simulink model "structure_implement"  (R2026b)
settings: Solver=VariableStepAuto
undefined symbols (not defined in the file or in its folder): DiscIntNeverNeededParam, Ts
settings Model: Creator=aomar  LastModifiedBy=aomar

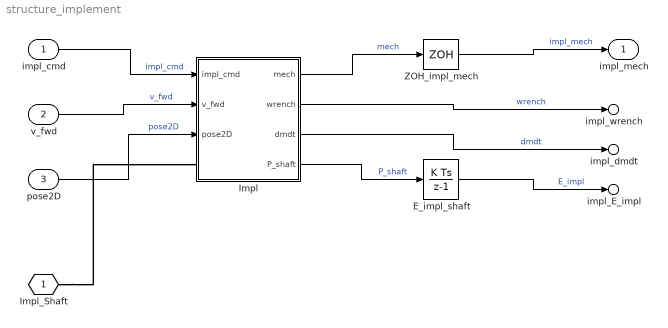
== system structure_implement ==
  impl_cmd : Inport  OutDataTypeStr=Bus: Bus_ImplementCmd  SampleTime=Ts.ctrl
  v_fwd : Inport  Port=2
  pose2D : Inport  Port=3
  E_impl_shaft : DiscreteIntegrator  gainval=1  SampleTime=Ts.base  ICPrevOutput=DiscIntNeverNeededParam  ICPrevScaledInput=DiscIntNeverNeededParam
  Impl : Subsystem  Variant=on
  ZOH_impl_mech : ZeroOrderHold  SampleTime=Ts.ctrl
  Impl_Shaft : PMIOPort  Side=Left  ConnectionType=Connection: foundation.mechanical.rotational.rotational
  impl_mech : Outport  OutDataTypeStr=Bus: Bus_ImplMechState  SampleTime=Ts.ctrl
  impl_wrench : Outport  Port=2  PortName=impl  Element=wrench
  impl_dmdt : Outport  Port=2  PortName=impl  Element=dmdt
  impl_E_impl : Outport  Port=2  PortName=impl  Element=E_impl
  wires:
  impl_cmd/1 -> Impl/1(impl_cmd)  "impl_cmd"
  v_fwd/1 -> Impl/2(v_fwd)  "v_fwd"
  pose2D/1 -> Impl/3(pose2D)  "pose2D"
  Impl/1(mech) -> ZOH_impl_mech/1  "mech"
  Impl/2(wrench) -> impl_wrench/1  "wrench"
  Impl/3(dmdt) -> impl_dmdt/1  "dmdt"
  Impl/4(P_shaft) -> E_impl_shaft/1  "P_shaft"
  ZOH_impl_mech/1 -> impl_mech/1  "impl_mech"
  E_impl_shaft/1 -> impl_E_impl/1  "E_impl"
  connections:
  Impl_Shaft/RConn1 -- Impl/LConn1

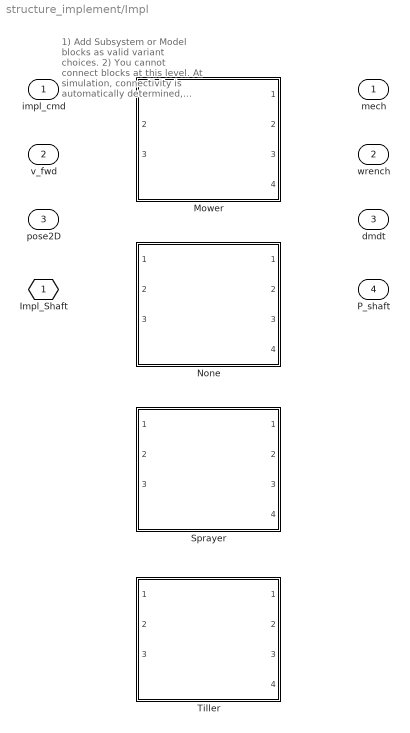
== system structure_implement/Impl ==
  note: 1) Add Subsystem or Model blocks as valid variant choices.
      | 2) You cannot connect blocks at this level. At simulation, connectivity is automatically
      | determined, based on the active variant and port name matching.
  impl_cmd : Inport  OutDataTypeStr=Bus: Bus_ImplementCmd
  v_fwd : Inport  Port=2
  pose2D : Inport  Port=3
  Mower : Subsystem  VariantControl=VC_IMPL == 1  ReferencedSubsystem=structure_impl_mower
  None : Subsystem  VariantControl=VC_IMPL == 0  ReferencedSubsystem=structure_impl_none
  Sprayer : Subsystem  VariantControl=VC_IMPL == 3  ReferencedSubsystem=structure_impl_sprayer
  Tiller : Subsystem  VariantControl=VC_IMPL == 2  ReferencedSubsystem=structure_impl_tiller
  Impl_Shaft : PMIOPort  Side=Left  ConnectionType=Connection: foundation.mechanical.rotational.rotational
  mech : Outport  OutDataTypeStr=Bus: Bus_ImplMechState
  wrench : Outport  Port=2
  dmdt : Outport  Port=3
  P_shaft : Outport  Port=4
